simulink model "TurnLightAct_fixed"  (R2023b)
settings: Solver=FixedStepDiscrete  StartTime=0.0  StopTime=10.0  FixedStep=0.01  RelTol=1e-3
undefined symbols (not defined in the file or in its folder): CtrlCmd, IoHwAb_TurnLightCtrlCmd_FL_Operation, IoHwAb_TurnLightCtrlCmd_FR_Operation, IoHwAb_TurnLightCtrlCmd_RL_Operation, IoHwAb_TurnLightCtrlCmd_RR_Operation
libraries: TurnLightActLib x4
settings Model: Creator=Wangjianwen  LastModifiedBy=123
settings SolverCC: AlgebraicLoopSolver=TrustRegion
settings DataIOCC: SaveFormat=StructureWithTime
settings OptimizationCC: DefaultParameterBehavior=Inlined  EnhancedBackFolding=on  PassReuseOutputArgsAs=Individual arguments  ZeroExternalMemoryAtStartup=off  ZeroInternalMemoryAtStartup=off  OptimizeBlockOrder=speed  DifferentSizesBufferReuse=on  OptimizationCustomize=off  EfficientTunableParamExpr=on
settings DebuggingCC: ParameterTunabilityLossMsg=error  UnconnectedInputMsg=warning  UnconnectedOutputMsg=warning  UnconnectedLineMsg=warning
settings HardwareCC: ProdLongLongMode=on
settings ModelReferenceCC: EnableRefExpFcnMdlSchedulingChecks=on  ModelReferenceNumInstancesAllowed=Single
settings SFSimCC: MATLABDynamicMemAlloc=off
settings RTWCC: Description=AUTOSAR  SystemTargetFile=autosar.tlc  GenCodeOnly=on  TemplateMakefile=ert_default_tmf  DataTypeReplacement=CDataTypesFixedWidth  DLArmComputeVersion=19.05
settings CodeAppCC: ForceParamTrailComments=on  IgnoreCustomStorageClasses=off  OperatorAnnotations=on  SimulinkDataObjDesc=on  SFDataObjDesc=on  InsertBlockDesc=on
settings STFCustomTargetCC: MultiwordLength=256  ParMdlRefBuildCompliant=on  CompOptLevelCompliant=on  IncludeMdlTerminateFcn=off  CombineOutputUpdateFcns=on  SuppressErrorStatus=on  ERTCustomFileBanners=on  SupportNonFinite=off  SupportComplex=off  SupportContinuousTime=off  SupportNonInlinedSFcns=off  RemoveResetFunc=on  MATLABClassNameForMDSCustomization=Simulink.SoftwareTarget.ERTCustomization  AutosarCompliant=on  UseToolchainInfoCompliant=on  LookupTableObjectStructAxisOrder=2,1,3,4,...  LUTObjectStructOrderEvenSpacing=Size,Table,Breakpoints  SystemTargetFile=autosar.tlc
settings ERTTargetCC: TargetLangStandard=C99 (ISO)  ConcurrentExecutionCompliant=off  IncludeMdlTerminateFcn=off  SuppressErrorStatus=on  SupportNonFinite=off  SupportComplex=off  ModelStepFunctionPrototypeControlCompliant=off  CPPClassGenCompliant=off  AutosarCompliant=on  LookupTableObjectStructAxisOrder=2,1,3,4,...  LUTObjectStructOrderEvenSpacing=Size,Table,Breakpoints  InlinedParameterPlacement=NonHierarchical  ERTCustomFileTemplate=example_file_process.tlc  BooleanTrueId=TRUE  BooleanFalseId=FALSE

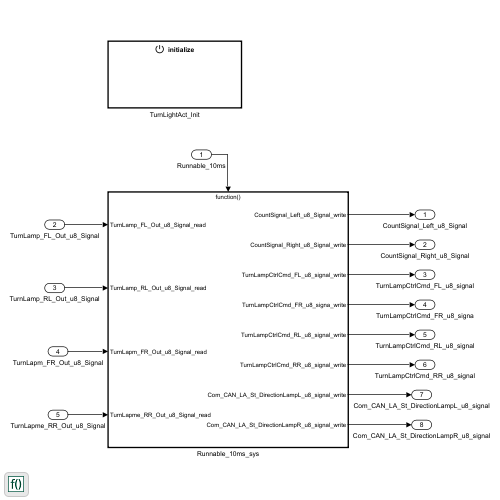
[thumbnail: Simulink's stored preview of the top-level diagram]
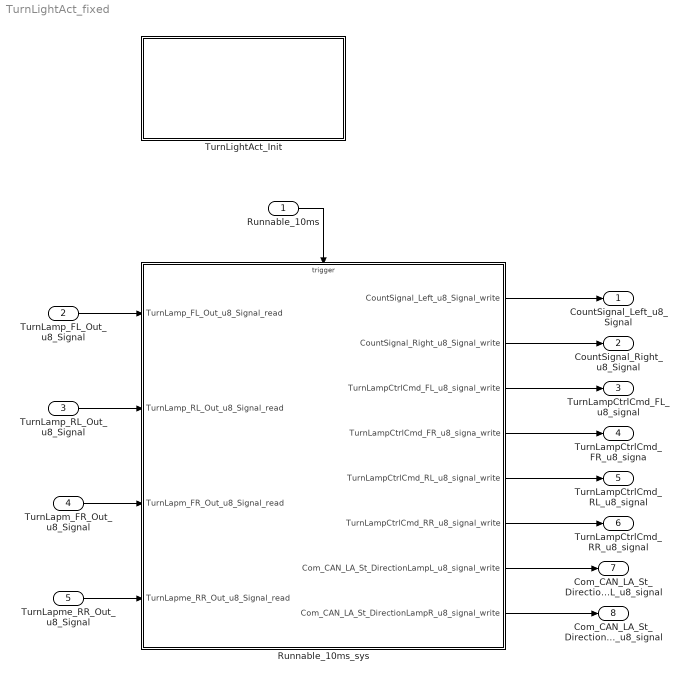
== system TurnLightAct_fixed ==
  Runnable_10ms : Inport  SampleTime=0.01  OutputFunctionCall=on
  TurnLamp_FL_Out_u8_Signal : Inport  Port=2  OutDataTypeStr=uint8  PortDimensions=1
  TurnLamp_RL_Out_u8_Signal : Inport  Port=3  OutDataTypeStr=uint8  PortDimensions=1
  TurnLapm_FR_Out_u8_Signal : Inport  Port=4  OutDataTypeStr=uint8  PortDimensions=1
  TurnLapme_RR_Out_u8_Signal : Inport  Port=5  OutDataTypeStr=uint8  PortDimensions=1
  Runnable_10ms_sys : Subsystem
  TurnLightAct_Init : Subsystem
  CountSignal_Left_u8_Signal : Outport  OutDataTypeStr=uint8  PortDimensions=1
  CountSignal_Right_u8_Signal : Outport  Port=2  OutDataTypeStr=uint8  PortDimensions=1
  TurnLampCtrlCmd_FL_u8_signal : Outport  Port=3  OutDataTypeStr=uint8  PortDimensions=1
  TurnLampCtrlCmd_FR_u8_signa : Outport  Port=4  OutDataTypeStr=uint8  PortDimensions=1
  TurnLampCtrlCmd_RL_u8_signal : Outport  Port=5  OutDataTypeStr=uint8  PortDimensions=1
  TurnLampCtrlCmd_RR_u8_signal : Outport  Port=6  OutDataTypeStr=uint8  PortDimensions=1
  Com_CAN_LA_St_DirectionLampL_u8_signal : Outport  Port=7  OutDataTypeStr=uint8  PortDimensions=1
  Com_CAN_LA_St_DirectionLampR_u8_signal : Outport  Port=8  OutDataTypeStr=uint8  PortDimensions=1
  wires:
  TurnLamp_FL_Out_u8_Signal/1 -> Runnable_10ms_sys/1(TurnLamp_FL_Out_u8_Signal_read)
  TurnLamp_RL_Out_u8_Signal/1 -> Runnable_10ms_sys/2(TurnLamp_RL_Out_u8_Signal_read)
  TurnLapm_FR_Out_u8_Signal/1 -> Runnable_10ms_sys/3(TurnLapm_FR_Out_u8_Signal_read)
  TurnLapme_RR_Out_u8_Signal/1 -> Runnable_10ms_sys/4(TurnLapme_RR_Out_u8_Signal_read)
  Runnable_10ms_sys/1(CountSignal_Left_u8_Signal_write) -> CountSignal_Left_u8_Signal/1
  Runnable_10ms_sys/2(CountSignal_Right_u8_Signal_write) -> CountSignal_Right_u8_Signal/1
  Runnable_10ms_sys/3(TurnLampCtrlCmd_FL_u8_signal_write) -> TurnLampCtrlCmd_FL_u8_signal/1
  Runnable_10ms_sys/4(TurnLampCtrlCmd_FR_u8_signa_write) -> TurnLampCtrlCmd_FR_u8_signa/1
  Runnable_10ms_sys/5(TurnLampCtrlCmd_RL_u8_signal_write) -> TurnLampCtrlCmd_RL_u8_signal/1
  Runnable_10ms_sys/6(TurnLampCtrlCmd_RR_u8_signal_write) -> TurnLampCtrlCmd_RR_u8_signal/1
  Runnable_10ms/1 -> Runnable_10ms_sys/Trigger
  Runnable_10ms_sys/7(Com_CAN_LA_St_DirectionLampL_u8_signal_write) -> Com_CAN_LA_St_DirectionLampL_u8_signal/1
  Runnable_10ms_sys/8(Com_CAN_LA_St_DirectionLampR_u8_signal_write) -> Com_CAN_LA_St_DirectionLampR_u8_signal/1

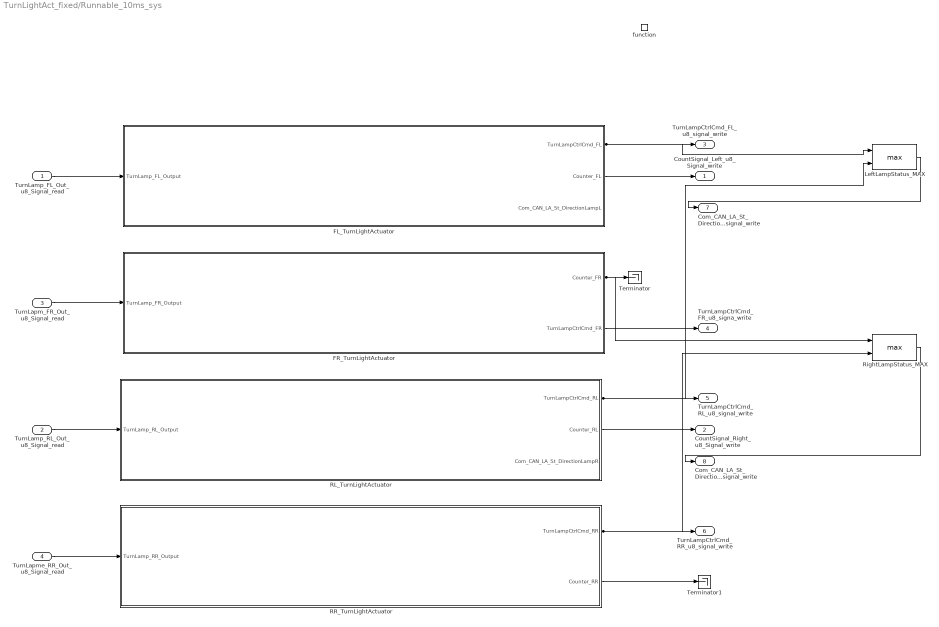
== system TurnLightAct_fixed/Runnable_10ms_sys ==
  TurnLamp_FL_Out_u8_Signal_read : Inport
  TurnLamp_RL_Out_u8_Signal_read : Inport  Port=2
  TurnLapm_FR_Out_u8_Signal_read : Inport  Port=3
  TurnLapme_RR_Out_u8_Signal_read : Inport  Port=4
  function : TriggerPort  TriggerType=function-call  VariantControl=(inherit)  SampleTimeType=periodic  SampleTime=-1
  FL_TurnLightActuator : Subsystem
  FR_TurnLightActuator : Subsystem
  LeftLampStatus_MAX : MinMax  Function=max  Inputs=2
  RL_TurnLightActuator : Subsystem
  RR_TurnLightActuator : Subsystem
  RightLampStatus_MAX : MinMax  Function=max  Inputs=2
  Terminator : Terminator
  Terminator1 : Terminator
  CountSignal_Left_u8_Signal_write : Outport
      settings: EnsureOutportIsVirtual=on
  CountSignal_Right_u8_Signal_write : Outport  Port=2
      settings: EnsureOutportIsVirtual=on
  TurnLampCtrlCmd_FL_u8_signal_write : Outport  Port=3
      settings: EnsureOutportIsVirtual=on
  TurnLampCtrlCmd_FR_u8_signa_write : Outport  Port=4
      settings: EnsureOutportIsVirtual=on
  TurnLampCtrlCmd_RL_u8_signal_write : Outport  Port=5
      settings: EnsureOutportIsVirtual=on
  TurnLampCtrlCmd_RR_u8_signal_write : Outport  Port=6
      settings: EnsureOutportIsVirtual=on
  Com_CAN_LA_St_DirectionLampL_u8_signal_write : Outport  Port=7
      settings: EnsureOutportIsVirtual=on
  Com_CAN_LA_St_DirectionLampR_u8_signal_write : Outport  Port=8
      settings: EnsureOutportIsVirtual=on
  wires:
  TurnLamp_FL_Out_u8_Signal_read/1 -> FL_TurnLightActuator/1(TurnLamp_FL_Output)
  TurnLamp_RL_Out_u8_Signal_read/1 -> RL_TurnLightActuator/1(TurnLamp_RL_Output)
  TurnLapm_FR_Out_u8_Signal_read/1 -> FR_TurnLightActuator/1(TurnLamp_FR_Output)
  TurnLapme_RR_Out_u8_Signal_read/1 -> RR_TurnLightActuator/1(TurnLamp_RR_Output)
  FL_TurnLightActuator/2(Counter_FL) -> CountSignal_Left_u8_Signal_write/1
  RL_TurnLightActuator/2(Counter_RL) -> CountSignal_Right_u8_Signal_write/1
  FL_TurnLightActuator/1(TurnLampCtrlCmd_FL) -> TurnLampCtrlCmd_FL_u8_signal_write/1, LeftLampStatus_MAX/1
  FR_TurnLightActuator/2(TurnLampCtrlCmd_FR) -> TurnLampCtrlCmd_FR_u8_signa_write/1
  RL_TurnLightActuator/1(TurnLampCtrlCmd_RL) -> TurnLampCtrlCmd_RL_u8_signal_write/1, LeftLampStatus_MAX/2
  RR_TurnLightActuator/1(TurnLampCtrlCmd_RR) -> TurnLampCtrlCmd_RR_u8_signal_write/1, RightLampStatus_MAX/2
  RR_TurnLightActuator/2(Counter_RR) -> Terminator1/1
  FR_TurnLightActuator/1(Counter_FR) -> Terminator/1, RightLampStatus_MAX/1
  LeftLampStatus_MAX/1 -> Com_CAN_LA_St_DirectionLampL_u8_signal_write/1
  RightLampStatus_MAX/1 -> Com_CAN_LA_St_DirectionLampR_u8_signal_write/1

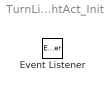
== system TurnLightAct_fixed/TurnLightAct_Init ==
  Event Listener : EventListener  EventName=reset

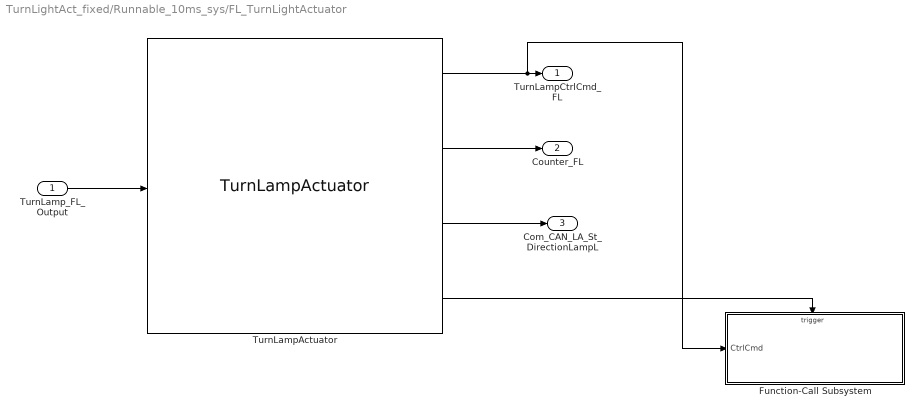
== system TurnLightAct_fixed/Runnable_10ms_sys/FL_TurnLightActuator ==
  TurnLamp_FL_Output : Inport
  Function-Call Subsystem : Subsystem  TreatAsAtomicUnit=on
  TurnLampActuator : TurnLightActLib/TurnLampActuator  SystemSampleTime=-1  VariantActivationTime=update diagram  Latency=0  AutoFrameSizeCalculation=off
  TurnLampCtrlCmd_FL : Outport
  Counter_FL : Outport  Port=2
  Com_CAN_LA_St_DirectionLampL : Outport  Port=3
  wires:
  TurnLamp_FL_Output/1 -> TurnLampActuator/1
  TurnLampActuator/2 -> Counter_FL/1
  TurnLampActuator/3 -> Com_CAN_LA_St_DirectionLampL/1
  TurnLampActuator/4 -> Function-Call Subsystem/Trigger
  TurnLampActuator/1 -> Function-Call Subsystem/1(CtrlCmd), TurnLampCtrlCmd_FL/1

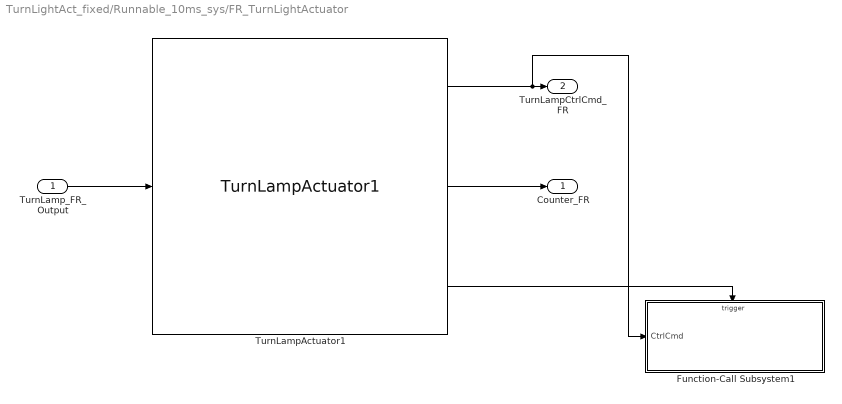
== system TurnLightAct_fixed/Runnable_10ms_sys/FR_TurnLightActuator ==
  TurnLamp_FR_Output : Inport
  Function-Call Subsystem1 : Subsystem  TreatAsAtomicUnit=on
  TurnLampActuator1 : TurnLightActLib/TurnLampActuator1  SystemSampleTime=-1  VariantActivationTime=update diagram  Latency=0  AutoFrameSizeCalculation=off
  Counter_FR : Outport
  TurnLampCtrlCmd_FR : Outport  Port=2
  wires:
  TurnLampActuator1/2 -> Counter_FR/1
  TurnLamp_FR_Output/1 -> TurnLampActuator1/1
  TurnLampActuator1/3 -> Function-Call Subsystem1/Trigger
  TurnLampActuator1/1 -> Function-Call Subsystem1/1(CtrlCmd), TurnLampCtrlCmd_FR/1

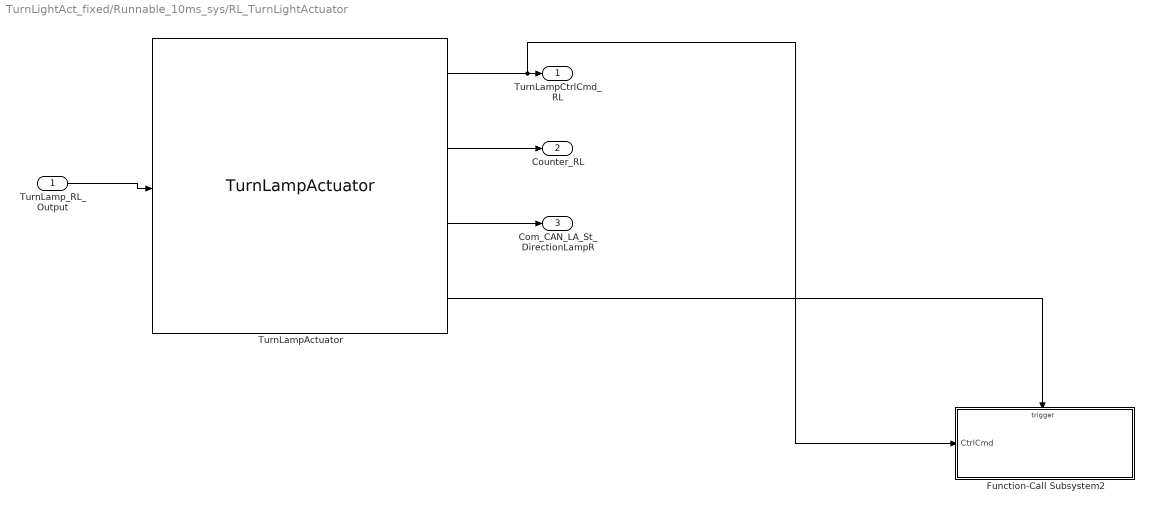
== system TurnLightAct_fixed/Runnable_10ms_sys/RL_TurnLightActuator ==
  TurnLamp_RL_Output : Inport
  Function-Call Subsystem2 : Subsystem  TreatAsAtomicUnit=on
  TurnLampActuator : TurnLightActLib/TurnLampActuator  SystemSampleTime=-1  VariantActivationTime=update diagram  Latency=0  AutoFrameSizeCalculation=off
  TurnLampCtrlCmd_RL : Outport
  Counter_RL : Outport  Port=2
  Com_CAN_LA_St_DirectionLampR : Outport  Port=3
  wires:
  TurnLamp_RL_Output/1 -> TurnLampActuator/1
  TurnLampActuator/1 -> Function-Call Subsystem2/1(CtrlCmd), TurnLampCtrlCmd_RL/1
  TurnLampActuator/2 -> Counter_RL/1
  TurnLampActuator/3 -> Com_CAN_LA_St_DirectionLampR/1
  TurnLampActuator/4 -> Function-Call Subsystem2/Trigger

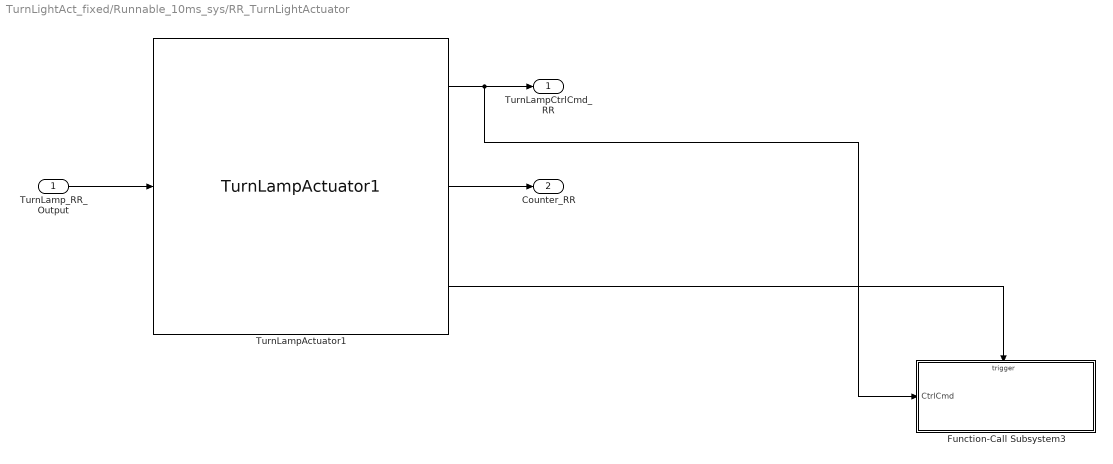
== system TurnLightAct_fixed/Runnable_10ms_sys/RR_TurnLightActuator ==
  TurnLamp_RR_Output : Inport
  Function-Call Subsystem3 : Subsystem  TreatAsAtomicUnit=on
  TurnLampActuator1 : TurnLightActLib/TurnLampActuator1  SystemSampleTime=-1  VariantActivationTime=update diagram  Latency=0  AutoFrameSizeCalculation=off
  TurnLampCtrlCmd_RR : Outport
  Counter_RR : Outport  Port=2
  wires:
  TurnLampActuator1/2 -> Counter_RR/1
  TurnLamp_RR_Output/1 -> TurnLampActuator1/1
  TurnLampActuator1/3 -> Function-Call Subsystem3/Trigger
  TurnLampActuator1/1 -> Function-Call Subsystem3/1(CtrlCmd), TurnLampCtrlCmd_RR/1

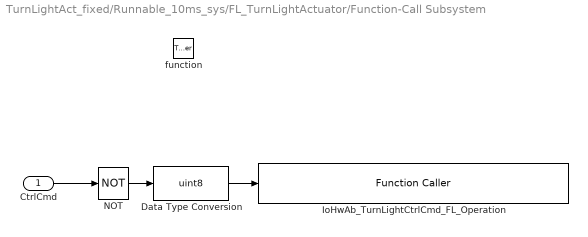
== system TurnLightAct_fixed/Runnable_10ms_sys/FL_TurnLightActuator/Function-Call Subsystem ==
  CtrlCmd : Inport
  function : TriggerPort  TriggerType=function-call  VariantControl=Variant
  Data Type Conversion : DataTypeConversion  OutDataTypeStr=uint8  SaturateOnIntegerOverflow=off  RndMeth=Floor
  IoHwAb_TurnLightCtrlCmd_FL_Operation : FunctionCaller  FunctionPrototype=IoHwAb_TurnLightCtrlCmd_FL_Operation(CtrlCmd)  InputArgumentSpecifications=uint8(1)
  NOT : Logic  Operator=NOT  IconShape=distinctive  AllPortsSameDT=off  OutDataTypeStr=boolean
  wires:
  CtrlCmd/1 -> NOT/1
  NOT/1 -> Data Type Conversion/1
  Data Type Conversion/1 -> IoHwAb_TurnLightCtrlCmd_FL_Operation/1

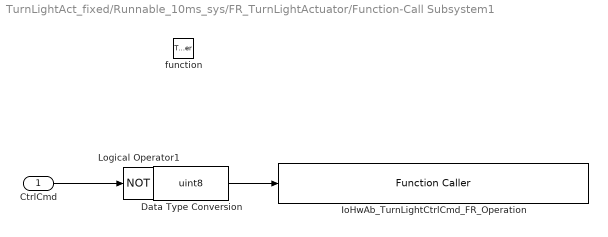
== system TurnLightAct_fixed/Runnable_10ms_sys/FR_TurnLightActuator/Function-Call Subsystem1 ==
  CtrlCmd : Inport
  function : TriggerPort  TriggerType=function-call  VariantControl=Variant
  Data Type Conversion : DataTypeConversion  OutDataTypeStr=uint8  SaturateOnIntegerOverflow=off  RndMeth=Floor
  IoHwAb_TurnLightCtrlCmd_FR_Operation : FunctionCaller  FunctionPrototype=IoHwAb_TurnLightCtrlCmd_FR_Operation(CtrlCmd)  InputArgumentSpecifications=uint8(1)
  Logical Operator1 : Logic  Operator=NOT  IconShape=distinctive  AllPortsSameDT=off  OutDataTypeStr=boolean
  wires:
  Logical Operator1/1 -> Data Type Conversion/1
  CtrlCmd/1 -> Logical Operator1/1
  Data Type Conversion/1 -> IoHwAb_TurnLightCtrlCmd_FR_Operation/1

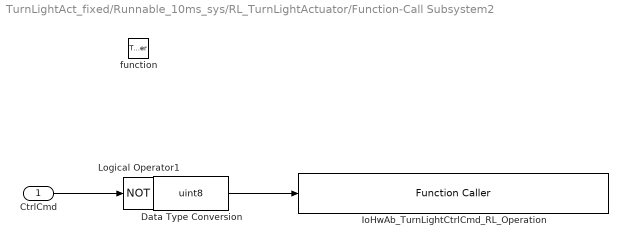
== system TurnLightAct_fixed/Runnable_10ms_sys/RL_TurnLightActuator/Function-Call Subsystem2 ==
  CtrlCmd : Inport
  function : TriggerPort  TriggerType=function-call  VariantControl=Variant
  Data Type Conversion : DataTypeConversion  OutDataTypeStr=uint8  SaturateOnIntegerOverflow=off  RndMeth=Floor
  IoHwAb_TurnLightCtrlCmd_RL_Operation : FunctionCaller  FunctionPrototype=IoHwAb_TurnLightCtrlCmd_RL_Operation(CtrlCmd)  InputArgumentSpecifications=uint8(1)
  Logical Operator1 : Logic  Operator=NOT  IconShape=distinctive  AllPortsSameDT=off  OutDataTypeStr=boolean
  wires:
  Logical Operator1/1 -> Data Type Conversion/1
  CtrlCmd/1 -> Logical Operator1/1
  Data Type Conversion/1 -> IoHwAb_TurnLightCtrlCmd_RL_Operation/1

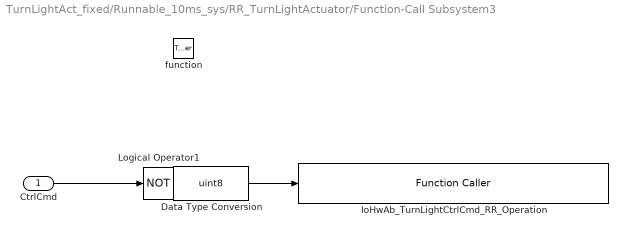
== system TurnLightAct_fixed/Runnable_10ms_sys/RR_TurnLightActuator/Function-Call Subsystem3 ==
  CtrlCmd : Inport
  function : TriggerPort  TriggerType=function-call  VariantControl=Variant
  Data Type Conversion : DataTypeConversion  OutDataTypeStr=uint8  SaturateOnIntegerOverflow=off  RndMeth=Floor
  IoHwAb_TurnLightCtrlCmd_RR_Operation : FunctionCaller  FunctionPrototype=IoHwAb_TurnLightCtrlCmd_RR_Operation(CtrlCmd)  InputArgumentSpecifications=uint8(1)
  Logical Operator1 : Logic  Operator=NOT  IconShape=distinctive  AllPortsSameDT=off  OutDataTypeStr=boolean
  wires:
  Logical Operator1/1 -> Data Type Conversion/1
  CtrlCmd/1 -> Logical Operator1/1
  Data Type Conversion/1 -> IoHwAb_TurnLightCtrlCmd_RR_Operation/1
